simulink subsystem "Subsys_GFolConv_OuterCtrl_NoCtrl"  (R2023b)
settings: Solver=VariableStepAuto  StartTime=0.0  StopTime=10.0  RelTol=1e-3
model mask{T_s_ctrl=1e-3, datatype='double'}
  mask prompts: T_s_ctrl "Controller sample time [s]"; datatype "Signal data type"
libraries: simulink x1
settings Model: Creator=winkens  LastModifiedBy=a.och
settings SolverCC: AlgebraicLoopSolver=TrustRegion
settings OptimizationCC: ReuseModelBlockBuffer=off
settings DebuggingCC: UnconnectedInputMsg=warning  UnconnectedOutputMsg=warning  UnconnectedLineMsg=warning
settings ModelReferenceCC: EnableRefExpFcnMdlSchedulingChecks=on
settings RTWCC: DLArmComputeVersion=19.05

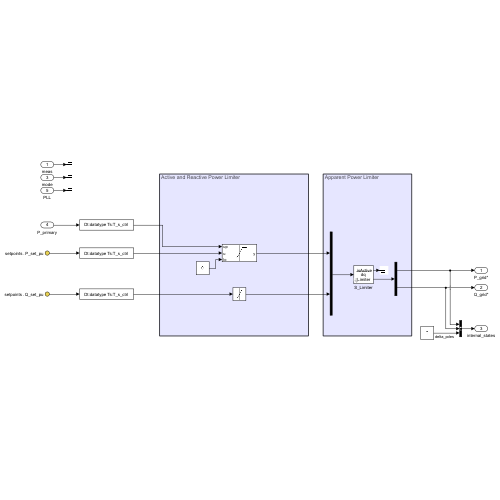
[thumbnail: Simulink's stored preview of the top-level diagram]
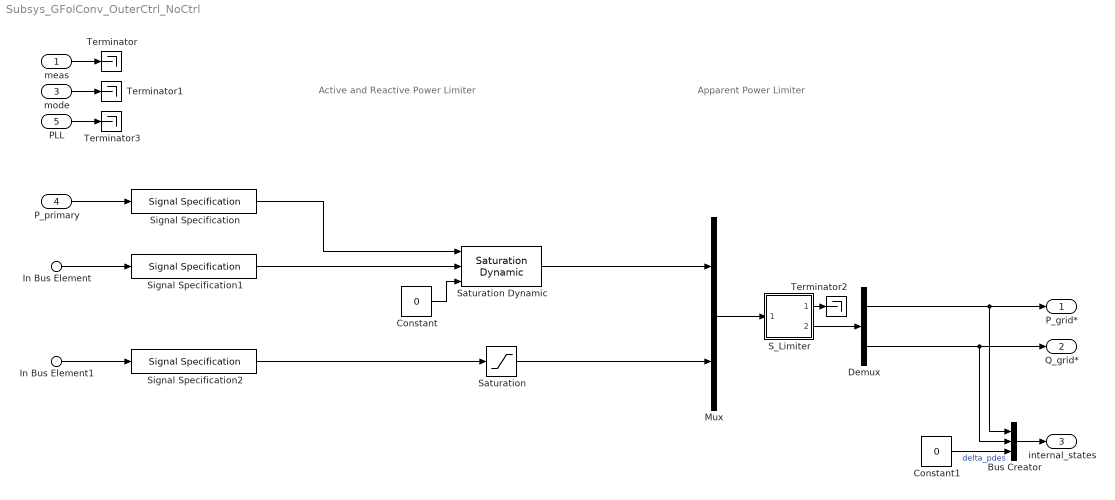
== system Subsys_GFolConv_OuterCtrl_NoCtrl ==
  note: Active and Reactive Power Limiter
  note: Apparent Power Limiter
  meas : Inport
  In Bus Element : Inport  Port=2  PortName=setpoints  Element=P_set_pu
  In Bus Element1 : Inport  Port=2  PortName=setpoints  Element=Q_set_pu
  mode : Inport  Port=3
  P_primary : Inport  Port=4
  PLL : Inport  Port=5
  Bus Creator : BusCreator  Inputs=3
  Constant : Constant  Value=0  OutDataTypeStr=datatype
  Constant1 : Constant  Value=0
  Demux : Demux  Outputs=2
  Mux : Mux  Inputs=2
  S_Limiter : Subsystem  ReferencedSubsystem=dq_Limiter  X_dq_max=1  datatype=datatype
  Saturation : Saturate  UpperLimit=1  LowerLimit=-1
  Saturation Dynamic : simulink/Discontinuities/Saturation Dynamic  OutMin=[]  OutMax=[]  OutDataTypeStr=Inherit: Same as second input  OutDataType=fixdt(1, 16)  OutScaling=2^-10  DoSatur=off
  Signal Specification : SignalSpecification  OutDataTypeStr=datatype  SampleTime=T_s_ctrl
  Signal Specification1 : SignalSpecification  OutDataTypeStr=datatype  SampleTime=T_s_ctrl
  Signal Specification2 : SignalSpecification  OutDataTypeStr=datatype  SampleTime=T_s_ctrl
  Terminator{,1..3} (4 alike) : Terminator
  P_grid* : Outport
  Q_grid* : Outport  Port=2
  internal_states : Outport  Port=3
  wires:
  Saturation Dynamic/1 -> Mux/1
  S_Limiter/2 -> Demux/1
  S_Limiter/1 -> Terminator2/1
  Mux/1 -> S_Limiter/1
  Saturation/1 -> Mux/2
  Demux/2 -> Bus Creator/2, Q_grid*/1
  Constant/1 -> Saturation Dynamic/3
  P_primary/1 -> Signal Specification/1
  Demux/1 -> P_grid*/1, Bus Creator/1
  In Bus Element/1 -> Signal Specification1/1
  In Bus Element1/1 -> Signal Specification2/1
  Bus Creator/1 -> internal_states/1
  mode/1 -> Terminator1/1
  meas/1 -> Terminator/1
  PLL/1 -> Terminator3/1
  Signal Specification/1 -> Saturation Dynamic/1
  Signal Specification1/1 -> Saturation Dynamic/2
  Signal Specification2/1 -> Saturation/1
  Constant1/1 -> Bus Creator/3  "delta_pdes"
